simulink model "obstacle_sensor_V1"  (R2025b)
settings: Solver=VariableStepAuto  StartTime=0.0  StopTime=10.0  RelTol=1e-3
undefined symbols (not defined in the file): floorsize, magnitude, rr_collide, rr_stop
libraries: simulink x4
settings Model: Creator=AORUS  LastModifiedBy=AORUS

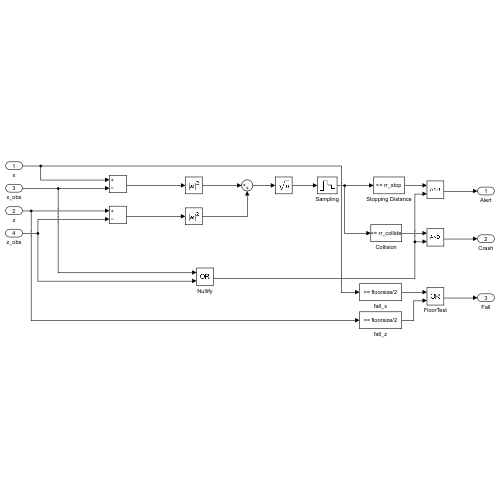
[thumbnail: Simulink's stored preview of the top-level diagram]
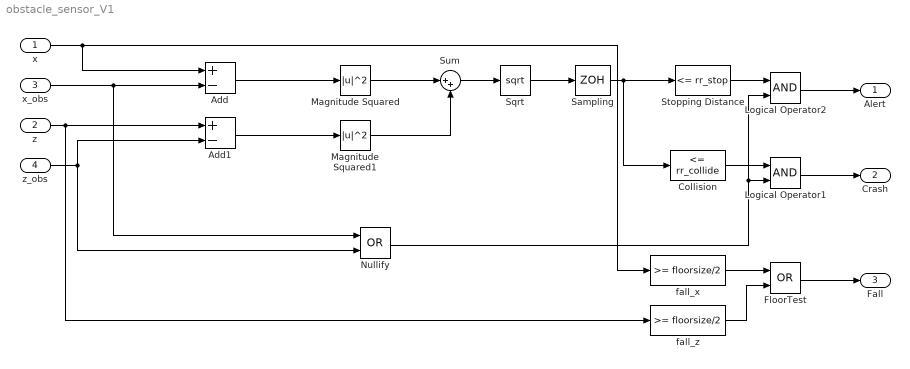
== system obstacle_sensor_V1 ==
  x : Inport
  z : Inport  Port=2
  x_obs : Inport  Port=3
  z_obs : Inport  Port=4
  Add : Sum  Inputs=+-
  Add1 : Sum  Inputs=+-
  Collision : simulink/Logic and Bit Operations/Compare To Constant  relop=<=  const=rr_collide  OutDataTypeStr=boolean
  FloorTest : Logic  Operator=OR  AllPortsSameDT=off  OutDataTypeStr=boolean
  Logical Operator1 : Logic  AllPortsSameDT=off  OutDataTypeStr=boolean
  Logical Operator2 : Logic  AllPortsSameDT=off  OutDataTypeStr=boolean
  Magnitude Squared : Math  Operator=magnitude^2
  Magnitude Squared1 : Math  Operator=magnitude^2
  Nullify : Logic  Operator=OR  AllPortsSameDT=off  OutDataTypeStr=boolean
  Sampling : ZeroOrderHold  SampleTime=0.25
  Sqrt : Sqrt
  Stopping Distance : simulink/Logic and Bit Operations/Compare To Constant  relop=<=  const=rr_stop  OutDataTypeStr=boolean
  Sum : Sum  Inputs=|++
  fall_x : simulink/Logic and Bit Operations/Compare To Constant  relop=>=  const=floorsize/2  OutDataTypeStr=boolean
  fall_z : simulink/Logic and Bit Operations/Compare To Constant  relop=>=  const=floorsize/2  OutDataTypeStr=boolean
  Alert : Outport
  Crash : Outport  Port=2
  Fall : Outport  Port=3
  wires:
  x/1 -> fall_x/1, Add/1
  fall_x/1 -> FloorTest/1
  FloorTest/1 -> Fall/1
  z_obs/1 -> Nullify/2, Add1/2
  Logical Operator1/1 -> Crash/1
  z/1 -> fall_z/1, Add1/1
  x_obs/1 -> Nullify/1, Add/2
  Collision/1 -> Logical Operator1/1
  Magnitude Squared/1 -> Sum/1
  Magnitude Squared1/1 -> Sum/2
  Logical Operator2/1 -> Alert/1
  Sum/1 -> Sqrt/1
  Add/1 -> Magnitude Squared/1
  Nullify/1 -> Logical Operator2/2, Logical Operator1/2
  Stopping Distance/1 -> Logical Operator2/1
  Sampling/1 -> Collision/1, Stopping Distance/1
  Sqrt/1 -> Sampling/1
  fall_z/1 -> FloorTest/2
  Add1/1 -> Magnitude Squared1/1
